simulink model "control_holist"  (R2024b)
settings: Solver=VariableStepAuto  StartTime=0.0  StopTime=10.0  RelTol=1e-3
libraries: slpidlib x2
settings Model: Creator=Edy  LastModifiedBy=Edy

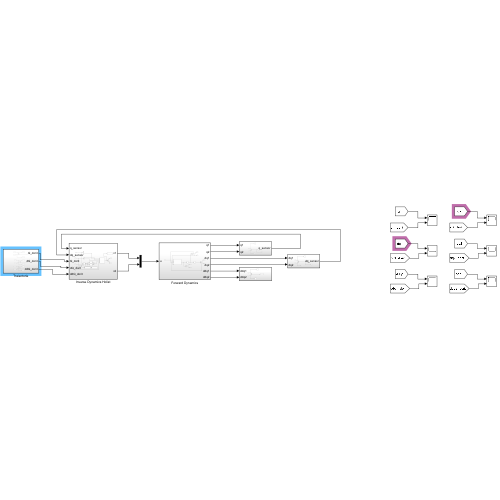
[thumbnail: Simulink's stored preview of the top-level diagram]
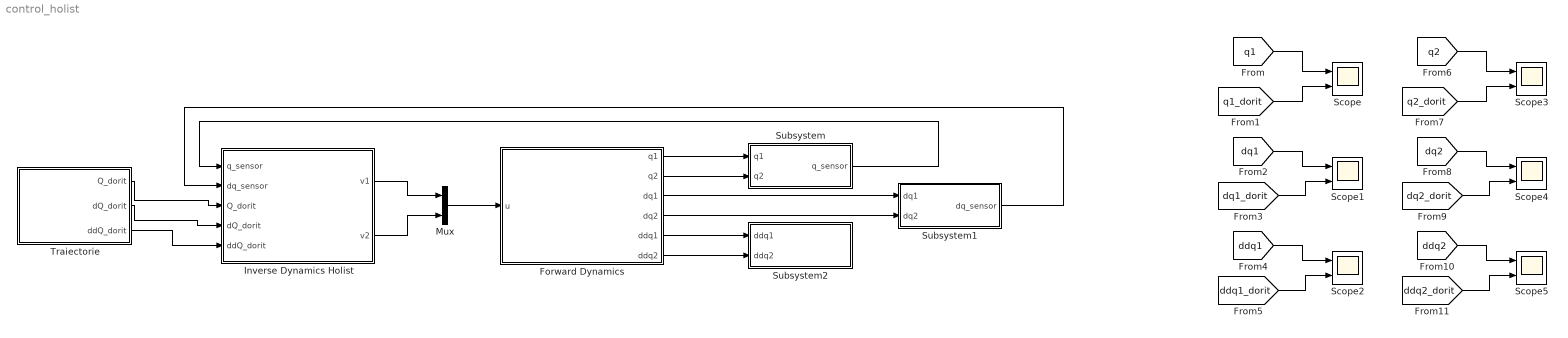
== system control_holist ==
  Forward Dynamics : Subsystem
  Inverse Dynamics Holist : Subsystem
  Mux : Mux  Inputs=2
  Scope{,1..5} (6 alike) : Scope  NumInputPorts=2
  Subsystem : Subsystem
  Subsystem1 : Subsystem
  Subsystem2 : Subsystem
  Traiectorie : Subsystem
  wires:
  Traiectorie/3(ddQ_dorit) -> Inverse Dynamics Holist/5(ddQ_dorit)
  Traiectorie/2(dQ_dorit) -> Inverse Dynamics Holist/4(dQ_dorit)
  Traiectorie/1(Q_dorit) -> Inverse Dynamics Holist/3(Q_dorit)
  Inverse Dynamics Holist/1(v1) -> Mux/1
  Inverse Dynamics Holist/2(v2) -> Mux/2
  Mux/1 -> Forward Dynamics/1(u)
  Forward Dynamics/1(q1) -> Subsystem/1(q1)
  Forward Dynamics/2(q2) -> Subsystem/2(q2)
  Forward Dynamics/3(dq1) -> Subsystem1/1(dq1)
  Forward Dynamics/4(dq2) -> Subsystem1/2(dq2)
  Forward Dynamics/5(ddq1) -> Subsystem2/1(ddq1)
  Forward Dynamics/6(ddq2) -> Subsystem2/2(ddq2)
  Subsystem/1(q_sensor) -> Inverse Dynamics Holist/1(q_sensor)
  Subsystem1/1(dq_sensor) -> Inverse Dynamics Holist/2(dq_sensor)
  [ddq1] -> Scope2/1
  [q2] -> Scope3/1
  [dq1_dorit] -> Scope1/2
  [ddq2] -> Scope5/1
  [ddq2_dorit] -> Scope5/2
  [ddq1_dorit] -> Scope2/2
  [dq2] -> Scope4/1
  [q1_dorit] -> Scope/2
  [q1] -> Scope/1
  [q2_dorit] -> Scope3/2
  [dq2_dorit] -> Scope4/2
  [dq1] -> Scope1/1

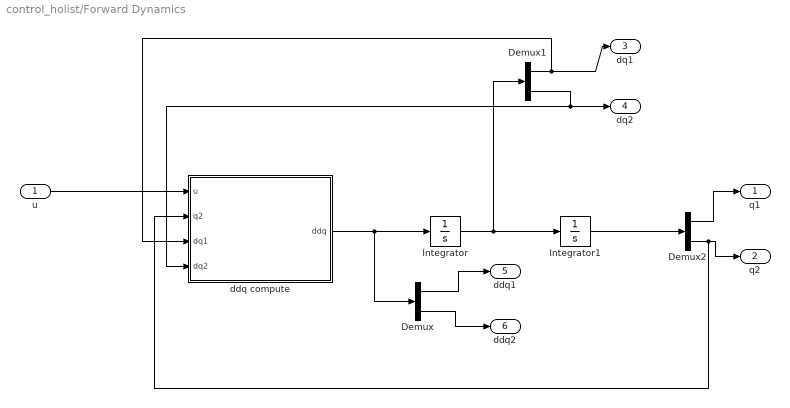
== system control_holist/Forward Dynamics ==
  u : Inport
  Demux : Demux  Outputs=2
  Demux1 : Demux  Outputs=2
  Demux2 : Demux  Outputs=2
  Integrator : Integrator
  Integrator1 : Integrator
  ddq compute : MATLAB Function  TreatAsAtomicUnit=on
  q1 : Outport
  q2 : Outport  Port=2
  dq1 : Outport  Port=3
  dq2 : Outport  Port=4
  ddq1 : Outport  Port=5
  ddq2 : Outport  Port=6
  wires:
  ddq compute/1(ddq) -> Demux/1, Integrator/1
  Integrator/1 -> Demux1/1, Integrator1/1
  Integrator1/1 -> Demux2/1
  Demux1/1 -> ddq compute/3(dq1), dq1/1
  Demux1/2 -> ddq compute/4(dq2), dq2/1
  u/1 -> ddq compute/1(u)
  Demux/1 -> ddq1/1
  Demux/2 -> ddq2/1
  Demux2/1 -> q1/1
  Demux2/2 -> ddq compute/2(q2), q2/1

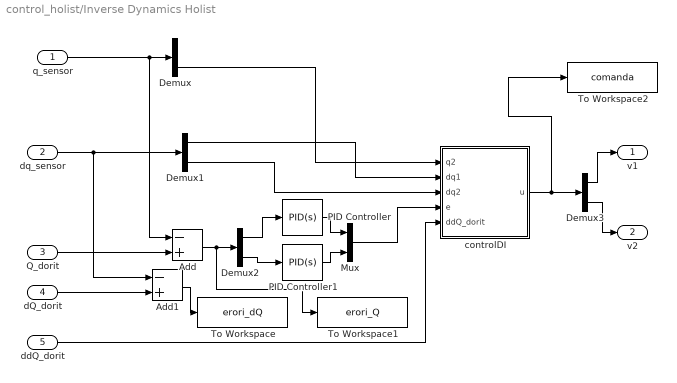
== system control_holist/Inverse Dynamics Holist ==
  q_sensor : Inport
  dq_sensor : Inport  Port=2
  Q_dorit : Inport  Port=3
  dQ_dorit : Inport  Port=4
  ddQ_dorit : Inport  Port=5
  Add : Sum  Inputs=-+
  Add1 : Sum  Inputs=-+
  Demux{,1..3} (4 alike) : Demux  Outputs=2
  Mux : Mux  Inputs=2
  PID Controller : slpidlib/PID Controller  Controller=PID  Form=Parallel  TimeDomain=Continuous-time  UseExternalTs=off  SampleTime=-1  IntegratorMethod=Forward Euler  FilterMethod=Forward Euler  ControllerParametersSource=internal  P=1  I=1  UseKiTs=off  D=0  UseExternalDerivativeSource=off  N=100  UseFilter=on  TunerSelectOption=Transfer Function Based (PID Tuner App)  InitialConditionSource=internal  InitialConditionForIntegrator=0  InitialConditionForFilter=0  DifferentiatorICPrevScaledInput=0  ExternalReset=none  TrackingMode=off  Kt=1  LimitOutput=off  SatLimitsSource=internal  UpperSaturationLimit=inf  LowerSaturationLimit=-inf  LinearizeAsGain=on  AntiWindupMode=none  Kb=1  LimitIntegrator=off  UpperIntegratorSaturationLimit=inf  LowerIntegratorSaturationLimit=-inf  POutMin=[]  POutMax=[]  IOutMin=[]  IOutMax=[]  DOutMin=[]  DOutMax=[]  NOutMin=[]  NOutMax=[]  SumOutMin=[]  SumOutMax=[]  SaturationOutMin=[]  SaturationOutMax=[]  PParamMin=[]  PParamMax=[]  IParamMin=[]  IParamMax=[]  DParamMin=[]  DParamMax=[]  NParamMin=[]  NParamMax=[]  KbParamMin=[]  KbParamMax=[]  KtParamMin=[]  KtParamMax=[]  KbOutMin=[]  KbOutMax=[]  KtOutMin=[]  KtOutMax=[]  IntegratorOutMin=[]  IntegratorOutMax=[]  FilterOutMin=[]  FilterOutMax=[]  SumI1OutMin=[]  SumI1OutMax=[]  SumI2OutMin=[]  SumI2OutMax=[]  SumI3OutMin=[]  SumI3OutMax=[]  SumI4OutMin=[]  SumI4OutMax=[]  SumDOutMin=[]  SumDOutMax=[]  DifferentiatorOutMin=[]  DifferentiatorOutMax=[]  FilterDiffOutCoefMin=[]  FilterDiffOutCoefMax=[]  ReciprocalOutMin=[]  ReciprocalOutMax=[]  SumDenOutMin=[]  SumDenOutMax=[]  SumNumOutMin=[]  SumNumOutMax=[]  DivideOutMin=[]  DivideOutMax=[]  UdiffTsProdOutMin=[]  UdiffTsProdOutMax=[]  NTsProdOutMin=[]  NTsProdOutMax=[]  UintegralTsProdOutMin=[]  UintegralTsProdOutMax=[]  UngainTsProdOutMin=[]  UngainTsProdOutMax=[]  ClampingZeroOutDataTypeStr=Inherit: Inherit via back propagation  ClampingZeroOutMin=[]  ClampingZeroOutMax=[]  FilterDenConstantOutDataTypeStr=Inherit: Inherit via back propagation  FilterDenConstantOutMin=[]  FilterDenConstantOutMax=[]  PCopyOutDataTypeStr=Inherit: Inherit via back propagation  PCopyOutMin=[]  PCopyOutMax=[]  NCopyOutDataTypeStr=Inherit: Inherit via back propagation  NCopyOutMin=[]  NCopyOutMax=[]  IntegratorContinuousStateAttributes=''  IntegratorStateMustResolveToSignalObject=off  IntegratorRTWStateStorageClass=Auto  FilterContinuousStateAttributes=''  FilterStateMustResolveToSignalObject=off  FilterRTWStateStorageClass=Auto  ParallelPVariant=InternalParameters  IdealPVariant=Disabled  IVariant=InternalParameters  DVariant=InternalParameters  IntegratorVariant=Continuous  SatVariant=Disabled  AWVariant=Passthrough  PCopyVariant=Disabled  TRVariant=Disabled  FdbkBlocksVariant=Forward  IdealPFdbkVariant=Disabled  SatFdbkVariant=Disabled  DerivativeFilterVariant=ContFilter  NVariant=InternalParameters  NCopyVariant=Disabled  FilterICVariant=InternalICsFilter  IntegratorICVariant=InternalICs  ExternalResetVariant=Disabled  TRSumVariant=Passthrough  SumFdbkVariant=Disabled  SumVariant=Sum_PID  TsampFilterVariant=InternalTs  TsampNgainVariant=Passthrough  TsampIntegralVariant=Disabled_SignalSpec  ExternalSaturationOutDataTypeStr=Inherit: Same as second input  DerivativeSourceVariant=ErrorSignal  PreIntVariant=InternalPreInt
  PID Controller1 : slpidlib/PID Controller  Controller=PID  Form=Parallel  TimeDomain=Continuous-time  UseExternalTs=off  SampleTime=-1  IntegratorMethod=Forward Euler  FilterMethod=Forward Euler  ControllerParametersSource=internal  P=1  I=1  UseKiTs=off  D=0  UseExternalDerivativeSource=off  N=100  UseFilter=on  TunerSelectOption=Transfer Function Based (PID Tuner App)  InitialConditionSource=internal  InitialConditionForIntegrator=0  InitialConditionForFilter=0  DifferentiatorICPrevScaledInput=0  ExternalReset=none  TrackingMode=off  Kt=1  LimitOutput=off  SatLimitsSource=internal  UpperSaturationLimit=inf  LowerSaturationLimit=-inf  LinearizeAsGain=on  AntiWindupMode=none  Kb=1  LimitIntegrator=off  UpperIntegratorSaturationLimit=inf  LowerIntegratorSaturationLimit=-inf  POutMin=[]  POutMax=[]  IOutMin=[]  IOutMax=[]  DOutMin=[]  DOutMax=[]  NOutMin=[]  NOutMax=[]  SumOutMin=[]  SumOutMax=[]  SaturationOutMin=[]  SaturationOutMax=[]  PParamMin=[]  PParamMax=[]  IParamMin=[]  IParamMax=[]  DParamMin=[]  DParamMax=[]  NParamMin=[]  NParamMax=[]  KbParamMin=[]  KbParamMax=[]  KtParamMin=[]  KtParamMax=[]  KbOutMin=[]  KbOutMax=[]  KtOutMin=[]  KtOutMax=[]  IntegratorOutMin=[]  IntegratorOutMax=[]  FilterOutMin=[]  FilterOutMax=[]  SumI1OutMin=[]  SumI1OutMax=[]  SumI2OutMin=[]  SumI2OutMax=[]  SumI3OutMin=[]  SumI3OutMax=[]  SumI4OutMin=[]  SumI4OutMax=[]  SumDOutMin=[]  SumDOutMax=[]  DifferentiatorOutMin=[]  DifferentiatorOutMax=[]  FilterDiffOutCoefMin=[]  FilterDiffOutCoefMax=[]  ReciprocalOutMin=[]  ReciprocalOutMax=[]  SumDenOutMin=[]  SumDenOutMax=[]  SumNumOutMin=[]  SumNumOutMax=[]  DivideOutMin=[]  DivideOutMax=[]  UdiffTsProdOutMin=[]  UdiffTsProdOutMax=[]  NTsProdOutMin=[]  NTsProdOutMax=[]  UintegralTsProdOutMin=[]  UintegralTsProdOutMax=[]  UngainTsProdOutMin=[]  UngainTsProdOutMax=[]  ClampingZeroOutDataTypeStr=Inherit: Inherit via back propagation  ClampingZeroOutMin=[]  ClampingZeroOutMax=[]  FilterDenConstantOutDataTypeStr=Inherit: Inherit via back propagation  FilterDenConstantOutMin=[]  FilterDenConstantOutMax=[]  PCopyOutDataTypeStr=Inherit: Inherit via back propagation  PCopyOutMin=[]  PCopyOutMax=[]  NCopyOutDataTypeStr=Inherit: Inherit via back propagation  NCopyOutMin=[]  NCopyOutMax=[]  IntegratorContinuousStateAttributes=''  IntegratorStateMustResolveToSignalObject=off  IntegratorRTWStateStorageClass=Auto  FilterContinuousStateAttributes=''  FilterStateMustResolveToSignalObject=off  FilterRTWStateStorageClass=Auto  ParallelPVariant=InternalParameters  IdealPVariant=Disabled  IVariant=InternalParameters  DVariant=InternalParameters  IntegratorVariant=Continuous  SatVariant=Disabled  AWVariant=Passthrough  PCopyVariant=Disabled  TRVariant=Disabled  FdbkBlocksVariant=Forward  IdealPFdbkVariant=Disabled  SatFdbkVariant=Disabled  DerivativeFilterVariant=ContFilter  NVariant=InternalParameters  NCopyVariant=Disabled  FilterICVariant=InternalICsFilter  IntegratorICVariant=InternalICs  ExternalResetVariant=Disabled  TRSumVariant=Passthrough  SumFdbkVariant=Disabled  SumVariant=Sum_PID  TsampFilterVariant=InternalTs  TsampNgainVariant=Passthrough  TsampIntegralVariant=Disabled_SignalSpec  ExternalSaturationOutDataTypeStr=Inherit: Same as second input  DerivativeSourceVariant=ErrorSignal  PreIntVariant=InternalPreInt
  To Workspace : ToWorkspace  VariableName=erori_dQ  SaveFormat=Timeseries  SampleTime=-1
  To Workspace1 : ToWorkspace  VariableName=erori_Q  SaveFormat=Timeseries  SampleTime=-1
  To Workspace2 : ToWorkspace  VariableName=comanda  SaveFormat=Timeseries  SampleTime=-1
  controlDI : MATLAB Function  TreatAsAtomicUnit=on
  v1 : Outport
  v2 : Outport  Port=2
  wires:
  q_sensor/1 -> Add/1, Demux/1
  Demux/2 -> controlDI/1(q2)
  dq_sensor/1 -> Add1/1, Demux1/1
  Q_dorit/1 -> Add/2
  dQ_dorit/1 -> Add1/2
  ddQ_dorit/1 -> controlDI/5(ddQ_dorit)
  Demux2/1 -> PID Controller/1
  Demux2/2 -> PID Controller1/1
  Add1/1 -> To Workspace/1
  Add/1 -> To Workspace1/1, Demux2/1
  PID Controller1/1 -> Mux/2
  PID Controller/1 -> Mux/1
  Demux1/1 -> controlDI/2(dq1)
  Demux1/2 -> controlDI/3(dq2)
  Mux/1 -> controlDI/4(e)
  controlDI/1(u) -> Demux3/1, To Workspace2/1
  Demux3/1 -> v1/1
  Demux3/2 -> v2/1

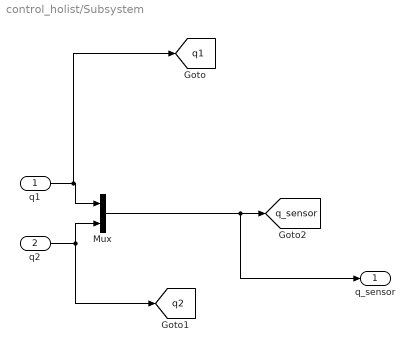
== system control_holist/Subsystem ==
  q1 : Inport
  q2 : Inport  Port=2
  Mux : Mux  Inputs=2
  q_sensor : Outport
  tag scope: q1=global, q2=global, q_sensor=global
  wires:
  q1/1 -> [q1], Mux/1
  q2/1 -> [q2], Mux/2
  Mux/1 -> q_sensor/1, [q_sensor]

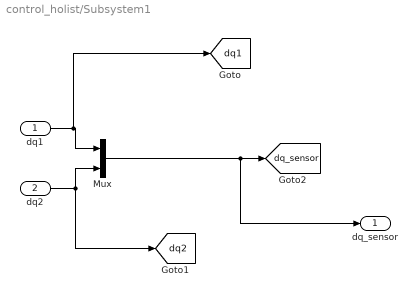
== system control_holist/Subsystem1 ==
  dq1 : Inport
  dq2 : Inport  Port=2
  Mux : Mux  Inputs=2
  dq_sensor : Outport
  tag scope: dq1=global, dq2=global, dq_sensor=global
  wires:
  dq1/1 -> [dq1], Mux/1
  dq2/1 -> [dq2], Mux/2
  Mux/1 -> dq_sensor/1, [dq_sensor]

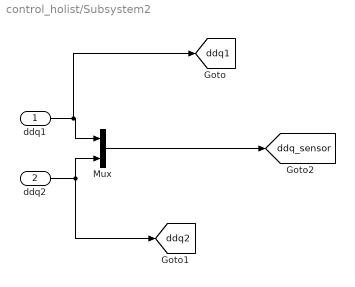
== system control_holist/Subsystem2 ==
  ddq1 : Inport
  ddq2 : Inport  Port=2
  Mux : Mux  Inputs=2
  tag scope: ddq1=global, ddq2=global, ddq_sensor=global
  wires:
  ddq1/1 -> [ddq1], Mux/1
  ddq2/1 -> [ddq2], Mux/2
  Mux/1 -> [ddq_sensor]

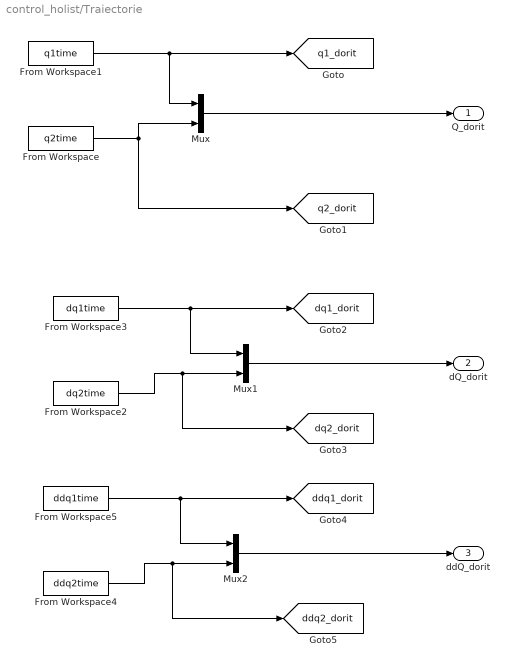
== system control_holist/Traiectorie ==
  From Workspace : FromWorkspace  VariableName=q2time
  From Workspace1 : FromWorkspace  VariableName=q1time
  From Workspace2 : FromWorkspace  VariableName=dq2time
  From Workspace3 : FromWorkspace  VariableName=dq1time
  From Workspace4 : FromWorkspace  VariableName=ddq2time
  From Workspace5 : FromWorkspace  VariableName=ddq1time
  Mux : Mux  Inputs=2
  Mux1 : Mux  Inputs=2
  Mux2 : Mux  Inputs=2
  Q_dorit : Outport
  dQ_dorit : Outport  Port=2
  ddQ_dorit : Outport  Port=3
  tag scope: ddq1_dorit=global, ddq2_dorit=global, dq1_dorit=global, dq2_dorit=global, q1_dorit=global, q2_dorit=global
  wires:
  Mux/1 -> Q_dorit/1
  From Workspace1/1 -> Mux/1, [q1_dorit]
  From Workspace/1 -> [q2_dorit], Mux/2
  From Workspace3/1 -> Mux1/1, [dq1_dorit]
  From Workspace2/1 -> [dq2_dorit], Mux1/2
  From Workspace4/1 -> [ddq2_dorit], Mux2/2
  From Workspace5/1 -> Mux2/1, [ddq1_dorit]
  Mux1/1 -> dQ_dorit/1
  Mux2/1 -> ddQ_dorit/1

== matlab function control_holist/Forward Dynamics/ddq compute ==
  data: u input; ddq output; q2 input; dq1 input; dq2 input
function ddq = forward_dynamics(u, q2, dq1, dq2)
    % =========================================================
    % 1. PARAMETRI STRUCTURA (R-T)
    % =========================================================
    m1 = 1;      
    m2 = 2;      
    l1 = 0.2;
    lc1 = 0.1;
    Izz1 = 3.68e-3;
    Izz2 = 7.366e-3;
    
    % =========================================================
    % 2. PARAMETRI MOTOR & TRANSMISIE
    % =========================================================
    % ATENTIE: J_t trebuie sa fie in kg*m^2! 
    % Daca in fisa e 72.8 g*cm^2, atunci e 72.8e-7 kg*m^2
    J_rotor = 72.8e-7; 
    
    i_r = 103;        % Raport reductor
    eta = 1/1.74;     % Randament (0.57)
    b_mot = 0.1;      % Frecare vascoasa la ax motor
    k_M = 27.3e-3;    % Constanta cuplu [Nm/A]
    R = 0.108;        % Rezistenta [Ohm]

    % Parametri Surub (Pt Cupla 2 - Translatie)
    pas_surub = 0.005; % [m]
    ht = pas_surub / (2*pi); % [m/rad] Constant de transmisie

    % =========================================================
    % 3. CALCUL FACTORI DE TRANSMISIE
    % =========================================================
    
    % Raportul de transformare a miscarii (Motor -> Brat)
    % Alpha 1: [rad_motor / rad_brat] = i_r
    % Alpha 2: [rad_motor / m_brat]   = i_r / ht
    alpha1 = i_r;
    alpha2 = i_r / ht;
    
    % Matricea de transformare (Diagonala)
    T_ratio = diag([alpha1, alpha2]); 

    % =========================================================
    % 4. DINAMICA BRATULUI (Mecanic)
    % =========================================================
    
    % Matricea de Inertie a Bratului M(q) - Specifica R-T
    M_brat = [m2*l1^2 + 2*m2*q2*l1 + m1*lc1^2 + m2*q2^2 + Izz1 + Izz2, 0; 
              0, m2];

    % Matricea Coriolis/Centrifugal C(q, dq)
    % Termeni specifici R-T (fara sin/cos la q2)
    Cn = [0, 0; 
         -m2*(l1 + q2), 0];
         
    B_coriolis_vec = [2*m2*(l1+q2); 
                      0];
                      
    % Fortele Nelineare Mecanice [Nm] si [N]
    N_mec = Cn*[dq1^2; dq2^2] + B_coriolis_vec*dq1*dq2;
    
    % Gravitatia (Zero in plan orizontal)
    G = [0; 0];

    % =========================================================
    % 5. ECUATIA TOTALA (Cuplaj Electric + Mecanic)
    % =========================================================
    % Ecuatia standard: M_total * ddq + N_total + B_total = Tau_generat
    
    % A. Inertia Totala (Brat + Rotor reflectat prin reductor)
    % Inertia rotorului se amplifica cu patratul raportului de transmisie!
    J_rotors_reflected = diag([J_rotor * alpha1^2 * eta, ...
                               J_rotor * alpha2^2 * eta]);
                           
    M_total = M_brat + J_rotors_reflected;
    
    % B. Forta generata de Tensiune (u)
    % Tau_mot = (k_M/R) * u ... apoi amplificat de reductor
    Gain_Force = (k_M / R) * eta;
    F_active = Gain_Force * T_ratio * u; 
    
    % C. Damping Total (Frecare Motor + Back-EMF) reflectat la brat
    % Back-EMF creeaza o franare proportionala cu viteza^2 (prin transmisie)
    Damp_coeff_motor = b_mot + (k_M^2 / R);
    
    % Matricea de damping reflectata
    B_total_mat = diag([Damp_coeff_motor * alpha1^2 * eta, ...
                        Damp_coeff_motor * alpha2^2 * eta]);
                    
    F_damping = B_total_mat * [dq1; dq2];
    
    % =========================================================
    % 6. CALCUL ACCELERATIE (ddq)
    % =========================================================
    
    % ddq = inv(M) * (Forte_Active - Nelinearitati - Damping - Gravitatie)
    ddq = M_total \ (F_active - N_mec - F_damping - G);

end

== matlab function control_holist/Inverse Dynamics Holist/controlDI ==
  data: q2 input; u output; dq1 input; dq2 input; e input; ddQ_dorit input
function u = controlul_DI(q2, dq1, dq2, e, ddQ_dorit)
    % Intrari conform schemei tale:
    % q2        : Pozitia liniara a cuplei 2 (metri)
    % dq1       : Viteza unghiulara cupla 1 (rad/s)
    % dq2       : Viteza liniara cupla 2 (m/s)
    % e         : Iesirea din blocurile PID externe (Corectia de acceleratie)
    % ddQ_dorit : Acceleratia din traiectorie
    
    % =========================================================
    % 1. PARAMETRI FIZICI (R-T cu Surub)
    % =========================================================
    m1 = 1;      
    m2 = 2;      
    l1 = 0.2;
    lc1 = 0.1;
    Izz1 = 3.68e-3;
    Izz2 = 7.366e-3;

    % Parametri Motor & Transmisie
    J_rotor = 72.8e-7; % [kg*m^2]
    b_mot   = 0.1;     % [Nms/rad]
    k_M     = 27.3e-3; % [Nm/A]
    R_coil  = 0.108;   % [Ohm]
    i_r     = 103;     % Raport reductor
    eta     = 1/1.74;  % Randament
    
    % Parametri Surub (Pt Cupla 2)
    pas_surub = 0.005; % [m]
    ht = pas_surub / (2*pi); % [m/rad]

    % =========================================================
    % 2. FACTORI DE CONVERSIE
    % =========================================================
    Gain_Volts_per_Nm = R_coil / k_M;
    
    % Conversie Sarcina -> Ax Motor
    Scale_J1 = 1 / (i_r * eta);         
    Scale_J2 = ht / (i_r * eta);        
    Gamma_Load = diag([Scale_J1, Scale_J2]);

    % =========================================================
    % 3. DINAMICA BRATULUI
    % =========================================================
    
    % Matricea de Inertie M(q) - Depinde doar de q2 (raza)
    M_brat = [m2*l1^2 + 2*m2*q2*l1 + m1*lc1^2 + m2*q2^2 + Izz1 + Izz2, 0; 
              0, m2];
          
    % Matricea Coriolis/Centrifugal
    Cn = [0, 0; -m2*(l1 + q2), 0];
    B_coriolis_vec = [2*m2*(l1+q2); 0];
    
    % Fortele nelineare
    N_brat = Cn*[dq1^2; dq2^2] + B_coriolis_vec*dq1*dq2;

    % =========================================================
    % 4. LEGEA DE COMANDA (Volti)
    % =========================================================
    
    % AICI E CHEIA: "acc_comanda" este acceleratia dorita + ce zice PID-ul (e)
    % Deoarece PID-ul tau este extern, el intra prin portul 'e'
    acc_comanda = ddQ_dorit + e;
    
    % Rapoarte transmisie (acceleratie motor vs brat)
    Alpha_acc_1 = i_r;
    Alpha_acc_2 = i_r / ht;
    
    % 1. Volti pentru Inertia Rotorului
    u_Jrot = Gain_Volts_per_Nm * J_rotor * [Alpha_acc_1 * acc_comanda(1); 
                                            Alpha_acc_2 * acc_comanda(2)];
                                        
    % 2. Volti pentru Inertia Bratului (M * a)
    u_Mbrat = Gain_Volts_per_Nm * Gamma_Load * M_brat * acc_comanda;
    
    % 3. Volti pentru Nelinearitati
    u_N = Gain_Volts_per_Nm * Gamma_Load * N_brat;
    
    % 4. Volti pentru Damping/Back-EMF
    dq_motor = [dq1 * Alpha_acc_1; 
                dq2 * Alpha_acc_2];
    u_Damping = (k_M + Gain_Volts_per_Nm * b_mot) * dq_motor;

    % Iesire
    u = u_Jrot + u_Mbrat + u_N + u_Damping;
end
